simulink model "WaveStar"  (R2018b)
settings: Solver=ode4  StartTime=0  StopTime=141.2  FixedStep=0.001  MaxStep=0.001  RelTol=1e-3  EnableMultiTasking=on
values from neighbouring files (symbols this model uses):
  cc = 10.0    (= 10)    [controller_init.m]
  kc = 0    [controller_init.m]
  L_AB = 0.412    [controller_init.m]
  L_AC = 0.2    [controller_init.m]
  mc = 0    [controller_init.m]
  McSat = inf    [controller_init.m]
  simu = simulationClass()    [wecSimInputFile.m]
  waves = waveClass('irregular')    [wecSimInputFile.m]
  xPcTs = 0.001    [controller_init.m]
undefined symbols (not defined in the file or in its folder): body, constraint, HPfreq, LPfreq, pto, X, Y, Z
libraries: nesl_utility x72, sm_lib x38, WECSim_Lib x7, simulink x2, vrlib x1
(part 3 of 4)

== system WaveStar/Float/Non-Hydro Body/Structure ==
  Total Force : Inport
  Body Properties : sm_lib/Body Elements/Solid  InertiaType=Custom  Mass=body.mass  MassUnits=kg  CenterOfMass=[0 0 0]  CenterOfMassUnits=m  MomentsOfInertia=body.momOfInertia  MomentsOfInertiaUnits=kg*m^2  ProductsOfInertia=[0 0 0]  ProductsOfInertiaUnits=kg*m^2  BasedOnType=Density  Density=1000  DensityUnits=kg/(m^3)  DoExposeReferenceFrame=on  SerializedFrames=<Frames/>  GraphicType=FromGeometry  MarkerShape=Sphere  MarkerSize=10  MarkerSizeUnits=m  GraphicVisPropType=SimpleVisualProperties  GraphicDiffuseColor=body.viz.color  GraphicSpecularColor=[0.5 0.5 0.5 1.0]  GraphicAmbientColor=[0.15 0.15 0.15 1.0]  GraphicEmissiveColor=[0.0 0.0 0.0 1.0]  GraphicShininess=75  GraphicOpacity=body.viz.opacity  GeometryShape=FromFile  RectangleSize=[1 1]  RectangleSizeUnits=m  BrickDimensions=[1 1 1]  BrickDimensionUnits=m  CylinderRadius=1  CylinderRadiusUnits=m  CylinderLength=1  CylinderLengthUnits=m  SphereRadius=1  SphereRadiusUnits=m  EllipsoidRadii=[1 1 1]  EllipsoidRadiiUnits=m  ExtrusionCrossSection=[1 1; -1 1; -1 -1; 1 -1]  ExtrusionCrossSectionUnits=m  ExtrusionLength=1  ExtrusionLengthUnits=m  PolygonNumSides=3  PolygonOuterRadius=1  PolygonOuterRadiusUnits=m  ExtGeomFileType=STL  ExtGeomFileName=geometry/Float.stl  ExtGeomFileUnits=m  RevolutionCrossSection=[1 1; 1 -1; 2 -1; 2 1]  RevolutionCrossSectionUnits=m  RevolutionExtent=Full  RevolutionAngle=180  RevolutionAngleUnits=deg
  External Force and Torque : sm_lib/Forces and Torques/External Force and Torque  ForceResolutionFrame=World  EnableForceX=off  EnableForceY=off  EnableForceZ=off  EnableForce=on  TorqueResolutionFrame=World  EnableTorqueX=off  EnableTorqueY=off  EnableTorqueZ=off  EnableTorque=on
  Motion Sensor : Subsystem
  Rigid Transform (Setup CG) : sm_lib/Frames and Transforms/Rigid Transform  TranslationMethod=Cartesian  TranslationStandardOffset=0  TranslationLengthUnit=m  TranslationStandardAxis=+Z  TranslationCartesianOffset=body.cg  TranslationROffset=0  TranslationROffsetUnits=m  TranslationZOffset=0  TranslationZOffsetUnits=m  TranslationThetaOffset=0  TranslationThetaOffsetUnits=deg  RotationMethod=None  RotationAngleUnits=rad  RotationStandardAxis=+Y  RotationAngle=0.05  RotationArbitraryAxis=[0.57735026918962584 0.57735026918962584 0.57735026918962584]  FollAlignAxisA=+X  BaseAlignAxisA=+Y  FollAlignAxisB=+Y  BaseAlignAxisB=+Z  RotationSequenceAxes=FollowerAxes  RotationSequence=XYX  RotationSequenceAngles=[0 0 0]  RotationSequenceAnglesUnits=deg  RotationMatrix=[1 0 0; 0 1 0; 0 0 1]
  Rigid Transform (Setup Initial Disp) : sm_lib/Frames and Transforms/Rigid Transform  TranslationMethod=Cartesian  TranslationStandardOffset=0  TranslationLengthUnit=m  TranslationStandardAxis=+Z  TranslationCartesianOffset=body.initDisp.initLinDisp  TranslationROffset=0  TranslationROffsetUnits=m  TranslationZOffset=0  TranslationZOffsetUnits=m  TranslationThetaOffset=0  TranslationThetaOffsetUnits=deg  RotationMethod=ArbitraryAxis  RotationAngleUnits=rad  RotationStandardAxis=+Y  RotationAngle=body.initDisp.initAngularDispAngle  RotationArbitraryAxis=body.initDisp.initAngularDispAxis  FollAlignAxisA=+X  BaseAlignAxisA=+Y  FollAlignAxisB=+Y  BaseAlignAxisB=+Z  RotationSequenceAxes=FollowerAxes  RotationSequence=XYX  RotationSequenceAngles=[0 0 0]  RotationSequenceAnglesUnits=deg  RotationMatrix=[1 0 0; 0 1 0; 0 0 1]
  Selector : Selector  InputPortWidth=6  IndexOptions=Index vector (dialog)  Indices=[1:3]  OutputSizes=1
  Selector1 : Selector  InputPortWidth=6  IndexOptions=Index vector (dialog)  Indices=[4:6]  OutputSizes=1
  Simulink-PS Converter1 : nesl_utility/Simulink-PS Converter  PhysicalDomain=network_engine_domain  SubClassName=ps_input  LeftPortType=input  RightPortType=output  PseudoPeriodic=off  Frequencies=[]  NoiseDistribution=none  NoiseParameters=[]  Unit=1  AffineConversion=off  FilteringAndDerivatives=zero  SimscapeFilterOrder=1  InputFilterTimeConstant=0.001  UdotUserProvided=1
  Simulink-PS Converter2 : nesl_utility/Simulink-PS Converter  PhysicalDomain=network_engine_domain  SubClassName=ps_input  LeftPortType=input  RightPortType=output  PseudoPeriodic=off  Frequencies=[]  NoiseDistribution=none  NoiseParameters=[]  Unit=1  AffineConversion=off  FilteringAndDerivatives=zero  SimscapeFilterOrder=1  InputFilterTimeConstant=0.001  UdotUserProvided=1
  World Frame : sm_lib/Frames and Transforms/World Frame
  Conn Free Surface : PMIOPort  Side=Right
  Response : Outport
  wires:
  Total Force/1 -> Selector1/1, Selector/1
  Selector/1 -> Simulink-PS Converter1/1
  Selector1/1 -> Simulink-PS Converter2/1
  Motion Sensor/1(Response) -> Response/1
  connections:
  External Force and Torque/LConn1 -- Simulink-PS Converter1/RConn1
  External Force and Torque/LConn2 -- Simulink-PS Converter2/RConn1
  Rigid Transform (Setup Initial Disp)/RConn1 -- Body Properties/RConn1 -- External Force and Torque/RConn1 -- Motion Sensor/RConn1
  Conn Free Surface/RConn1 -- Rigid Transform (Setup CG)/LConn1
  Rigid Transform (Setup Initial Disp)/LConn1 -- Rigid Transform (Setup CG)/RConn1
  World Frame/RConn1 -- Motion Sensor/LConn1

== system WaveStar/Float/Non-Hydro Body/Weight and Buoyancy ==
  Add1 : Sum  Inputs=+-
  Assignment (Add Net Bouyancy Force to Z-Direction) : Assignment  IndexOptions=Index vector (dialog)  Indices=3  OutputSizes=1
  Body Mass : Constant  Value=body.mass
  Constant1 : Constant  Value=[0 0 0 0 0 0]
  Gravity : Constant  Value=simu.g
  Product : Product
  Product1 : Product  Inputs=3
  Volume : Constant  Value=body.dispVol
  Water Density : Constant  Value=simu.rho
  Out1 : Outport
  wires:
  Add1/1 -> Assignment (Add Net Bouyancy Force to Z-Direction)/2
  Product1/1 -> Add1/2  "F_Buoyancy"
  Product/1 -> Add1/1  "F_Gravity"
  Water Density/1 -> Product1/1  "rho"
  Gravity/1 -> Product/1, Product1/2  "g"
  Volume/1 -> Product1/3  "Vol"
  Assignment (Add Net Bouyancy Force to Z-Direction)/1 -> Out1/1  "F_Restoring"
  Constant1/1 -> Assignment (Add Net Bouyancy Force to Z-Direction)/1
  Body Mass/1 -> Product/2  "m"

== system WaveStar/Controller/Linear/WECCCOMP Controller/lin2rot conversion ==
  float_accel_rot : Inport
  "motor_pos " : Inport  Port=2
  Axial Position : Selector  InputPortWidth=6  IndexOptions=Index vector (dialog)  Indices=[3]  OutputSizes=1
  Constant : Constant  Value=L_AC
  Differentiator with break frequency : DiscreteTransferFcn  Numerator=[1 -1]*2*2*pi*HPfreq.vel  Denominator=[(2+2*pi*HPfreq.vel*xPcTs) (2*pi*HPfreq.vel*xPcTs-2)]
  Divide : Product  Inputs=**
  First order LP filter : DiscreteTransferFcn  Numerator=[1 1]*xPcTs*2*pi*LPfreq.vel  Denominator=[(2+xPcTs*2*pi*LPfreq.vel) (xPcTs*2*pi*LPfreq.vel-2)]
  Linear2Angular Conversion : Subsystem
  Terminator : Terminator
  "float_accel " : Outport
  moment_arm : Outport  Port=2
  motor_vel : Outport  Port=3
  wires:
  "motor_pos "/1 -> Differentiator with break frequency/1, Axial Position/1
  Linear2Angular Conversion/2(moment_arm) -> moment_arm/1
  Axial Position/1 -> Linear2Angular Conversion/1(x_cyl)
  Linear2Angular Conversion/1(Theta) -> Terminator/1
  float_accel_rot/1 -> Divide/1
  Constant/1 -> Divide/2
  Divide/1 -> "float_accel "/1  "Angular Acceleration"
  Differentiator with break frequency/1 -> First order LP filter/1
  First order LP filter/1 -> motor_vel/1

== system WaveStar/Controller/Linear/WECCCOMP Controller/rot2lin conversion ==
  cmd_force_ref : Inport
  moment_arm : Inport  Port=2
  "Divide " : Product  Inputs=*/
  Gain : Gain  Gain=-1
  Multiply : Product  Inputs=**
  Saturation : Saturate  UpperLimit=McSat  LowerLimit=-McSat
  comand torque to measured torque dynamics : DiscreteTransferFcn  Numerator="[ 0.9821   -1.9618    0.9797]"  Denominator="[1.0000   -1.9978    0.9978]"
  cmd_force : Outport
  wires:
  "Divide "/1 -> cmd_force/1
  moment_arm/1 -> Multiply/2, "Divide "/2
  Saturation/1 -> Gain/1  "Mc_sat"
  Gain/1 -> "Divide "/1
  comand torque to measured torque dynamics/1 -> Saturation/1
  cmd_force_ref/1 -> Multiply/1
  Multiply/1 -> comand torque to measured torque dynamics/1

== system WaveStar/Controller/Rotary/lin2rot conversion/Linear2Angular Conversion ==
  x_cyl : Inport
  Divide => K (m) : Product  Inputs=*/
  MATLAB Function1 K [m] : MATLAB Function  TreatAsAtomicUnit=on
  MATLAB Function1 L_BC [m] : MATLAB Function  TreatAsAtomicUnit=on
  MATLAB Function1 Theta [rad] : MATLAB Function  TreatAsAtomicUnit=on
  MATLAB Function1 a_CAB [rad] : MATLAB Function  TreatAsAtomicUnit=on
  Theta : Outport
  moment_arm : Outport  Port=2
  wires:
  MATLAB Function1 L_BC [m]/1(y) -> [L_BC]
  [a_CAB] -> MATLAB Function1 Theta [rad]/1(u)
  MATLAB Function1 K [m]/1(y) -> Divide => K (m)/1
  [L_BC] -> MATLAB Function1 a_CAB [rad]/1(u)
  [L_BC] -> Divide => K (m)/2
  x_cyl/1 -> MATLAB Function1 L_BC [m]/1(u)
  Divide => K (m)/1 -> moment_arm/1
  MATLAB Function1 a_CAB [rad]/1(y) -> [a_CAB]
  [a_CAB] -> MATLAB Function1 K [m]/1(u)
  MATLAB Function1 Theta [rad]/1(y) -> Theta/1

== system WaveStar/Float/Hydrodynamic Body/B2B Subsystem/B2B ==
  CrossCoupling : Subsystem  mask{body=body}
      mask prompts: body "Body Number"
      mask help: This is used to
      mask init:
      | %In the initialization tab we place the code modifying the block
      | 
      | cb = gcb;
      | % position of initial blocks
      | set_param([cb '/vel1'],'Position',[200 1*50 240 (1*50+30)])
      | set_param([cb '/Mux1'], 'Position',[375 40 380 90])
      | set_param([cb '/vel'], 'Position',[410 59 440 71])
      | set_param([cb '/acc1'],'Position',[600 1*50 640 (1*50+30)])
      | set_param([cb '/Mux2'], 'Position',[775 40 780 90])
      | set_param([cb '/acc'], 'Position',[810 59 840 71])
      | 
      | % add/delete lines & blocks
      | newInputs = 0;
      | numbodies = body.bodyTotal;
      | iBod = 2;
      | while iBod < 100
      |     try 
      |         find_system([cb,'/vel',num2str(iBod)],'Type','Block');
      |         if iBod > numbodies
      |             %delete 'From' blocks and lines if bodynumber > total bodies
      |             delete_line(cb,['vel',num2str(iBod),'/1'],['Mux',num2str(1),'/',num2str(iBod)])
      |             delete_line(cb,['acc',num2str(iBod),'/1'],['Mux',num2str(2),'/',num2str(iBod)])
      |             delete_block([cb '/vel',num2str(iBod)])
      |             delete_block([cb '/acc',num2str(iBod)])
      |         end
      |     catch
      |         %set number of outputs for 'Mux Creator' blocks 
      |         if newInputs==0
      |             set_param([cb,'/Mux1'],'Inputs',num2str(numbodies))
      |             set_param([cb,'/Mux2'],'Inputs',num2str(numbodies))
      |         end
      |         if iBod <= numbodies
      |             newInputs = newInputs + 1;
      |             %add velocity 'From' block
      |             add_block('simulink/Signal Routing/From', [cb,'/vel',num2str(iBod)],'MakeNameUnique', 'on',...
      |             'Position',[200 iBod*50 240 (iBod*50+30)], 'BackgroundColor','green')
      |             h=[cb,'/vel',num2str(iBod)];
      |             responseName=['vel' num2str(iBod)];
      |             set_param(h,'GotoTag',responseName);
      |             %add acceleration 'From' block
      |             add_block('simulink/Signal Routing/From', [cb,'/acc',num2str(iBod)],'MakeNameUnique', 'on',...
      |             'Position',[600 iBod*50 640 (iBod*50+30)], 'BackgroundColor','green')
      |             h=[cb,'/acc',num2str(iBod)];
      |             responseName=['acc' num2str(iBod)];
      |             set_param(h,'GotoTag',responseName);
      |             %add lines
      |             add_line(cb,['vel',num2str(iBod),'/1'],['Mux',num2str(1),'/',num2str(iBod)])
      |             add_line(cb,['acc',num2str(iBod),'/1'],['Mux',num2str(2),'/',num2str(iBod)])
      |         else
      |             break
      |         end
      |     end
      |     iBod = iBod + 1;
      | end
      mask Callback body: %customsat_callback('input',gcb)
      mask DialogControl DescGroupVar Prompt: Coupling Block
      mask DialogControl DescTextVar Prompt: This block transfers the velocity and acceleration vectors between bodies allowing for the coupled hydrodynamic forces to be calculated.  This block should not be included if there is only one body or if the hydrodynamic coupling parameter is set to 'No' in the rigid body block.
  vel : Outport
  acc : Outport  Port=2
  wires:
  CrossCoupling/2(acc) -> acc/1
  CrossCoupling/1(vel) -> vel/1

== system WaveStar/Float/Hydrodynamic Body/B2B Subsystem/noB2B ==
  vel_in : Inport
  acc_in : Inport  Port=2
  vel : Outport
  acc : Outport  Port=2
  wires:
  acc_in/1 -> acc/1
  vel_in/1 -> vel/1  "x"

== system WaveStar/Float/Hydrodynamic Body/Hydrostatic Restoring Force Calculation/Linear and Nonlinear Restoring Force Variant Subsystem ==
  note: 1) Add Subsystem or Model blocks as valid variant choices.
      | 2) You cannot connect blocks at this level. At simulation, connectivity is automatically
      | determined, based on the active variant and port name matching.
  In1 : Inport
  In2 : Inport  Port=2
  "Linear Hydrostatic Restoring Force " : Subsystem  VariantControl=sv_linearHydro
  Nonlinear Hydrostatic Restoring Force : Subsystem  VariantControl=sv_nonlinearHydro
  Out1 : Outport

== system WaveStar/Float/Hydrodynamic Body/Morison Element and ViscousDampingForceCalculation/Morison Element Variant Subsystem ==
  note: 1) Add Subsystem or Model blocks as valid variant choices.
      | 2) You cannot connect blocks at this level. At simulation, connectivity is automatically
      | determined, based on the active variant and port name matching.
  displacement : Inport
  velocity : Inport  Port=2
  acceleration : Inport  Port=3
  time : Inport  Port=4
  Morison Element Off : Subsystem  VariantControl=sv_MEOff
  Morison Element On : Subsystem  Variant=on  VariantControl=sv_MEOn
  morison_force : Outport

== system WaveStar/Float/Hydrodynamic Body/Nonlinear Wave Elevation/Linear or Instantaneous Free Surface ==
  note: 1) Add Subsystem or Model blocks as valid variant choices.
      | 2) You cannot connect blocks at this level. At simulation, connectivity is automatically
      | determined, based on the active variant and port name matching.
  In1 : Inport
  In2 : Inport  Port=2
  "Instantaneous Water Free Surface  " : Subsystem  VariantControl=sv_instFS
  "Mean Water Free Surface " : Subsystem  VariantControl=sv_meanFS
  Out1 : Outport

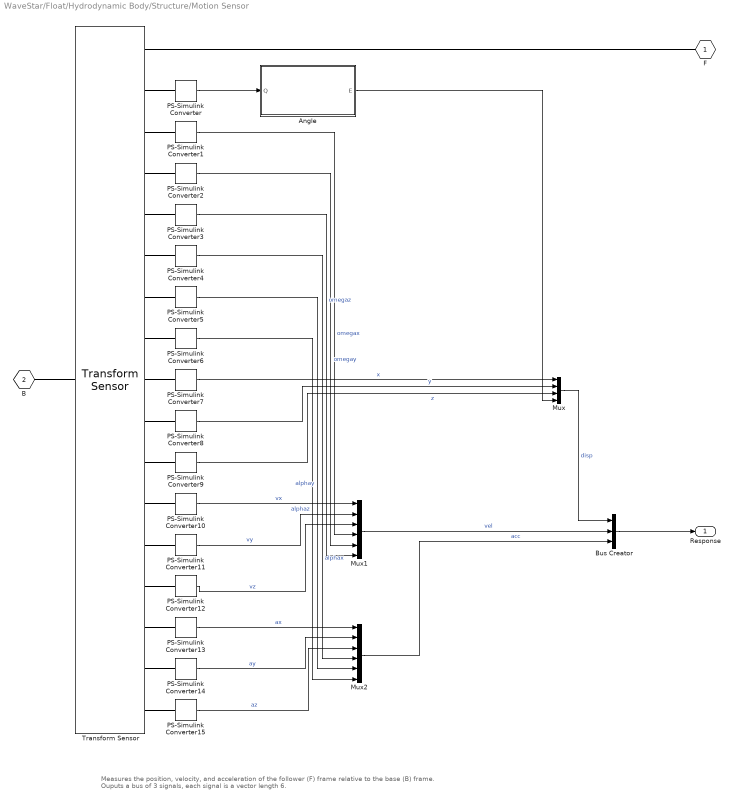
== system WaveStar/Float/Hydrodynamic Body/Structure/Motion Sensor ==
  note: Measures the position, velocity, and acceleration of the follower (F) frame relative to the base (B) frame.
      | Ouputs a bus of 3 signals, each signal is a vector length 6.
  Angle : MATLAB Function  TreatAsAtomicUnit=on
  Bus Creator : BusCreator  Inputs=3
  Mux : Mux
  Mux1 : Mux  Inputs=6
  Mux2 : Mux  Inputs=6
  PS-Simulink Converter{,1..15} (16 alike) : nesl_utility/PS-Simulink Converter  PhysicalDomain=network_engine_domain  SubClassName=ps_output  LeftPortType=input  RightPortType=output  PseudoPeriodic=off  Frequencies=[]  Unit=1  AffineConversion=off
  Transform Sensor : sm_lib/Frames and Transforms/Transform Sensor  MeasurementFrame=World  SenseAngle=off  SenseAxis=off  SenseAngle1=off  SenseAngle2=off  SenseAngle3=off  SenseQ=on  SenseR=off  SenseOmegaX=on  SenseOmegaY=on  SenseOmegaZ=on  SenseOmega1=off  SenseOmega2=off  SenseOmega3=off  SenseQDot=off  SenseRDot=off  SenseAlphaX=on  SenseAlphaY=on  SenseAlphaZ=on  SenseAlpha1=off  SenseAlpha2=off  SenseAlpha3=off  SenseQDDot=off  SenseRDDot=off  SenseX=on  SenseY=on  SenseZ=on  SenseRad=off  SenseAzim=off  SenseDist=off  SenseInc=off  SenseXDot=on  SenseYDot=on  SenseZDot=on  SenseRadDot=off  SenseAzimDot=off  SenseDistDot=off  SenseIncDot=off  SenseXDDot=on  SenseYDDot=on  SenseZDDot=on  SenseRadDDot=off  SenseAzimDDot=off  SenseDistDDot=off  SenseIncDDot=off
  F : PMIOPort  Side=Right
  B : PMIOPort  Port=2  Side=Left
  Response : Outport
  wires:
  PS-Simulink Converter/1 -> Angle/1(Q)
  PS-Simulink Converter4/1 -> Mux2/4  "alphax"
  PS-Simulink Converter10/1 -> Mux1/1  "vx"
  PS-Simulink Converter12/1 -> Mux1/3  "vz"
  PS-Simulink Converter13/1 -> Mux2/1  "ax"
  PS-Simulink Converter14/1 -> Mux2/2  "ay"
  Mux/1 -> Bus Creator/1  "disp"
  Mux1/1 -> Bus Creator/2  "vel"
  Mux2/1 -> Bus Creator/3  "acc"
  Angle/1(E) -> Mux/4
  PS-Simulink Converter7/1 -> Mux/1  "x"
  PS-Simulink Converter8/1 -> Mux/2  "y"
  PS-Simulink Converter9/1 -> Mux/3  "z"
  PS-Simulink Converter5/1 -> Mux2/5  "alphay"
  PS-Simulink Converter6/1 -> Mux2/6  "alphaz"
  PS-Simulink Converter1/1 -> Mux1/4  "omegax"
  PS-Simulink Converter2/1 -> Mux1/5  "omegay"
  PS-Simulink Converter11/1 -> Mux1/2  "vy"
  PS-Simulink Converter3/1 -> Mux1/6  "omegaz"
  PS-Simulink Converter15/1 -> Mux2/3  "az"
  Bus Creator/1 -> Response/1
  connections:
  Transform Sensor/RConn1 -- F/RConn1
  B/RConn1 -- Transform Sensor/LConn1
  Transform Sensor/RConn2 -- PS-Simulink Converter/LConn1
  PS-Simulink Converter15/LConn1 -- Transform Sensor/RConn17
  PS-Simulink Converter14/LConn1 -- Transform Sensor/RConn16
  PS-Simulink Converter13/LConn1 -- Transform Sensor/RConn15
  PS-Simulink Converter12/LConn1 -- Transform Sensor/RConn14
  PS-Simulink Converter11/LConn1 -- Transform Sensor/RConn13
  PS-Simulink Converter10/LConn1 -- Transform Sensor/RConn12
  PS-Simulink Converter9/LConn1 -- Transform Sensor/RConn11
  PS-Simulink Converter8/LConn1 -- Transform Sensor/RConn10
  PS-Simulink Converter7/LConn1 -- Transform Sensor/RConn9
  PS-Simulink Converter4/LConn1 -- Transform Sensor/RConn6
  PS-Simulink Converter5/LConn1 -- Transform Sensor/RConn7
  PS-Simulink Converter6/LConn1 -- Transform Sensor/RConn8
  PS-Simulink Converter1/LConn1 -- Transform Sensor/RConn3
  PS-Simulink Converter2/LConn1 -- Transform Sensor/RConn4
  PS-Simulink Converter3/LConn1 -- Transform Sensor/RConn5

== system WaveStar/Float/Hydrodynamic Body/Wave Diffraction and Excitation Force Calculation/Linear Wave Excitation Force Variant Subsystem ==
  note: 1) Add Subsystem or Model blocks as valid variant choices.
      | 2) You cannot connect blocks at this level. At simulation, connectivity is automatically
      | determined, based on the active variant and port name matching.
  Time : Inport
  Irregular Wave Excitation Force : Subsystem  VariantControl=sv_irregularWaves
  No Wave Excitation Force : Subsystem  VariantControl=sv_noWave
  Regular Wave Excitation Force : Subsystem  VariantControl=sv_regularWaves
  User Defined Wave Excitation Force : Subsystem  VariantControl=sv_udfWaves
  Linear Excitation : Outport

== system WaveStar/Float/Hydrodynamic Body/Wave Diffraction and Excitation Force Calculation/No Ramp Function ==
  Action Port : ActionPort  ActionType=else
  Constant : Constant
  R : Outport  InitialOutput=1
  wires:
  Constant/1 -> R/1

== system WaveStar/Float/Hydrodynamic Body/Wave Diffraction and Excitation Force Calculation/Nonlinear FK Force Variant Subsystem ==
  note: 1) Add Subsystem or Model blocks as valid variant choices.
      | 2) You cannot connect blocks at this level. At simulation, connectivity is automatically
      | determined, based on the active variant and port name matching.
  Time : Inport
  Displacement : Inport  Port=2
  WaveElv : Inport  Port=3
  No Nonlinear FroudeKrylov Force : Subsystem  VariantControl=sv_linearHydro
  With Nonlinear FroudeKrylov Force : Subsystem  TreatAsAtomicUnit=on  SystemSampleTime=simu.dtNL  VariantControl=sv_nonlinearHydro
  Nonlinear Excitation : Outport

== system WaveStar/Float/Hydrodynamic Body/Wave Diffraction and Excitation Force Calculation/Ramp Function ==
  Time : Inport
  Action Port : ActionPort  ActionType=then
  Add : Sum
  Add1 : Sum
  Constant : Constant  Value=1/2
  Constant1 : Constant
  Constant2 : Constant  Value=3*pi/2
  Constant3 : Constant  Value=pi
  Divide : Product  Inputs=*/
  Product : Product
  Product1 : Product
  Ramp Time : Constant  Value=simu.rampTime
  Sine Wave Function : Sin  TimeSource=Use external signal  SampleTime=0
  R : Outport
  wires:
  Divide/1 -> Product1/2  "frequency"
  Constant3/1 -> Divide/1
  Product1/1 -> Add1/1
  Add1/1 -> Sine Wave Function/1
  Constant2/1 -> Add1/2  "phase"
  Ramp Time/1 -> Divide/2  "t_ramp"
  Time/1 -> Product1/1  "t"
  Product/1 -> R/1
  Constant/1 -> Product/2
  Constant1/1 -> Add/1
  Sine Wave Function/1 -> Add/2
  Add/1 -> Product/1

== system WaveStar/Float/Hydrodynamic Body/Wave Radiation Forces Calculation/SS CI and Constant-Damping-CoeVariant Subsystem ==
  note: 1) Add Subsystem or Model blocks as valid variant choices.
      | 2) You cannot connect blocks at this level. At simulation, connectivity is automatically
      | determined, based on the active variant and port name matching.
  In1 : Inport
  In2 : Inport  Port=2
  Constant Coefficients : Subsystem  VariantControl=sv_constantCoeff
  Convolution Integral Calculation : Subsystem  VariantControl=sv_convolution
  "State-Space Calculation " : Subsystem  VariantControl=sv_stateSpace
  Out1 : Outport

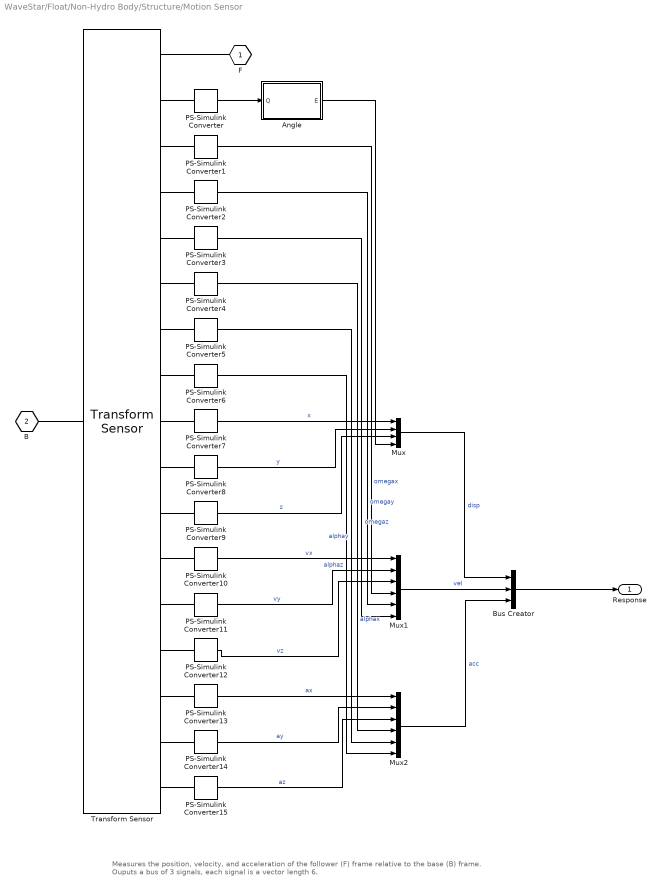
== system WaveStar/Float/Non-Hydro Body/Structure/Motion Sensor ==
  note: Measures the position, velocity, and acceleration of the follower (F) frame relative to the base (B) frame.
      | Ouputs a bus of 3 signals, each signal is a vector length 6.
  Angle : MATLAB Function  TreatAsAtomicUnit=on
  Bus Creator : BusCreator  Inputs=3
  Mux : Mux
  Mux1 : Mux  Inputs=6
  Mux2 : Mux  Inputs=6
  PS-Simulink Converter{,1..15} (16 alike) : nesl_utility/PS-Simulink Converter  PhysicalDomain=network_engine_domain  SubClassName=ps_output  LeftPortType=input  RightPortType=output  PseudoPeriodic=off  Frequencies=[]  Unit=1  AffineConversion=off
  Transform Sensor : sm_lib/Frames and Transforms/Transform Sensor  MeasurementFrame=World  SenseAngle=off  SenseAxis=off  SenseAngle1=off  SenseAngle2=off  SenseAngle3=off  SenseQ=on  SenseR=off  SenseOmegaX=on  SenseOmegaY=on  SenseOmegaZ=on  SenseOmega1=off  SenseOmega2=off  SenseOmega3=off  SenseQDot=off  SenseRDot=off  SenseAlphaX=on  SenseAlphaY=on  SenseAlphaZ=on  SenseAlpha1=off  SenseAlpha2=off  SenseAlpha3=off  SenseQDDot=off  SenseRDDot=off  SenseX=on  SenseY=on  SenseZ=on  SenseRad=off  SenseAzim=off  SenseDist=off  SenseInc=off  SenseXDot=on  SenseYDot=on  SenseZDot=on  SenseRadDot=off  SenseAzimDot=off  SenseDistDot=off  SenseIncDot=off  SenseXDDot=on  SenseYDDot=on  SenseZDDot=on  SenseRadDDot=off  SenseAzimDDot=off  SenseDistDDot=off  SenseIncDDot=off
  F : PMIOPort  Side=Right
  B : PMIOPort  Port=2  Side=Left
  Response : Outport
  wires:
  PS-Simulink Converter/1 -> Angle/1(Q)
  PS-Simulink Converter4/1 -> Mux2/4  "alphax"
  PS-Simulink Converter10/1 -> Mux1/1  "vx"
  PS-Simulink Converter12/1 -> Mux1/3  "vz"
  PS-Simulink Converter13/1 -> Mux2/1  "ax"
  PS-Simulink Converter14/1 -> Mux2/2  "ay"
  Mux/1 -> Bus Creator/1  "disp"
  Mux1/1 -> Bus Creator/2  "vel"
  Mux2/1 -> Bus Creator/3  "acc"
  Angle/1(E) -> Mux/4
  PS-Simulink Converter7/1 -> Mux/1  "x"
  PS-Simulink Converter8/1 -> Mux/2  "y"
  PS-Simulink Converter9/1 -> Mux/3  "z"
  PS-Simulink Converter5/1 -> Mux2/5  "alphay"
  PS-Simulink Converter6/1 -> Mux2/6  "alphaz"
  PS-Simulink Converter1/1 -> Mux1/4  "omegax"
  PS-Simulink Converter2/1 -> Mux1/5  "omegay"
  PS-Simulink Converter11/1 -> Mux1/2  "vy"
  PS-Simulink Converter3/1 -> Mux1/6  "omegaz"
  PS-Simulink Converter15/1 -> Mux2/3  "az"
  Bus Creator/1 -> Response/1
  connections:
  Transform Sensor/RConn1 -- F/RConn1
  B/RConn1 -- Transform Sensor/LConn1
  Transform Sensor/RConn2 -- PS-Simulink Converter/LConn1
  PS-Simulink Converter15/LConn1 -- Transform Sensor/RConn17
  PS-Simulink Converter14/LConn1 -- Transform Sensor/RConn16
  PS-Simulink Converter13/LConn1 -- Transform Sensor/RConn15
  PS-Simulink Converter12/LConn1 -- Transform Sensor/RConn14
  PS-Simulink Converter11/LConn1 -- Transform Sensor/RConn13
  PS-Simulink Converter10/LConn1 -- Transform Sensor/RConn12
  PS-Simulink Converter9/LConn1 -- Transform Sensor/RConn11
  PS-Simulink Converter8/LConn1 -- Transform Sensor/RConn10
  PS-Simulink Converter7/LConn1 -- Transform Sensor/RConn9
  PS-Simulink Converter4/LConn1 -- Transform Sensor/RConn6
  PS-Simulink Converter5/LConn1 -- Transform Sensor/RConn7
  PS-Simulink Converter6/LConn1 -- Transform Sensor/RConn8
  PS-Simulink Converter1/LConn1 -- Transform Sensor/RConn3
  PS-Simulink Converter2/LConn1 -- Transform Sensor/RConn4
  PS-Simulink Converter3/LConn1 -- Transform Sensor/RConn5

== system WaveStar/Controller/Linear/WECCCOMP Controller/lin2rot conversion/Linear2Angular Conversion ==
  x_cyl : Inport
  Divide => K (m) : Product  Inputs=*/
  MATLAB Function1 K [m] : MATLAB Function  TreatAsAtomicUnit=on
  MATLAB Function1 L_BC [m] : MATLAB Function  TreatAsAtomicUnit=on
  MATLAB Function1 Theta [rad] : MATLAB Function  TreatAsAtomicUnit=on
  MATLAB Function1 a_CAB [rad] : MATLAB Function  TreatAsAtomicUnit=on
  Theta : Outport
  moment_arm : Outport  Port=2
  wires:
  MATLAB Function1 L_BC [m]/1(y) -> [L_BC]
  [a_CAB] -> MATLAB Function1 Theta [rad]/1(u)
  MATLAB Function1 K [m]/1(y) -> Divide => K (m)/1
  [L_BC] -> MATLAB Function1 a_CAB [rad]/1(u)
  [L_BC] -> Divide => K (m)/2
  x_cyl/1 -> MATLAB Function1 L_BC [m]/1(u)
  Divide => K (m)/1 -> moment_arm/1
  MATLAB Function1 a_CAB [rad]/1(y) -> [a_CAB]
  [a_CAB] -> MATLAB Function1 K [m]/1(u)
  MATLAB Function1 Theta [rad]/1(y) -> Theta/1

== system WaveStar/Float/Hydrodynamic Body/B2B Subsystem/B2B/CrossCoupling ==
  note: CrossCoupling block is updated by its mask initialization, which is only called on when a simulation is run. 'From' blocks are automatically created and connected based on the number of bodies in the simulation.
  Mux1 : Mux  Inputs=2
  Mux2 : Mux  Inputs=2
  vel : Outport
  acc : Outport  Port=2
  wires:
  [acc2] -> Mux2/2
  Mux2/1 -> acc/1
  [acc1] -> Mux2/1
  [vel2] -> Mux1/2
  Mux1/1 -> vel/1
  [vel1] -> Mux1/1

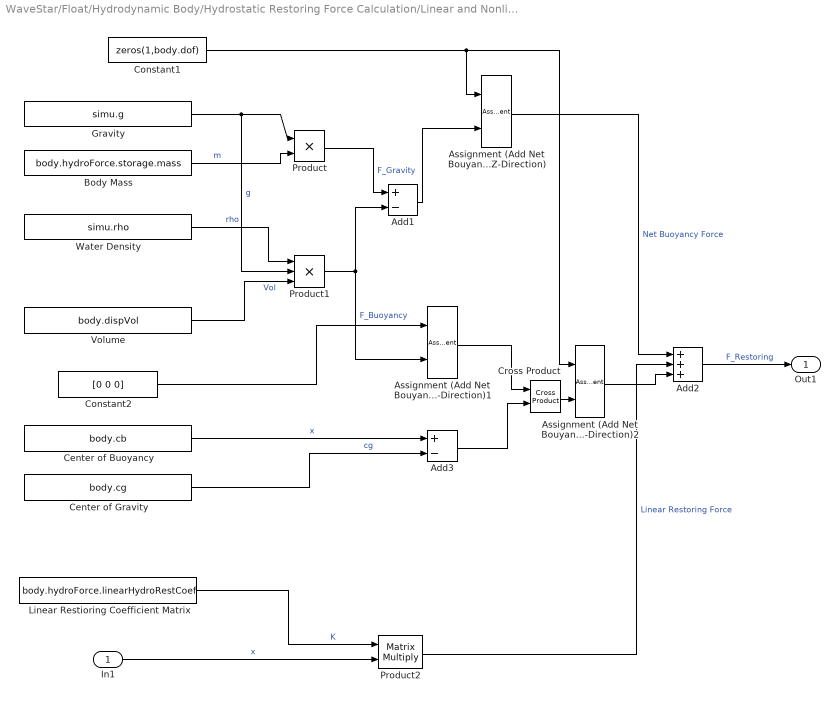
== system WaveStar/Float/Hydrodynamic Body/Hydrostatic Restoring Force Calculation/Linear and Nonlinear Restoring Force Variant Subsystem/Linear Hydrostatic Restoring Force  ==
  In1 : Inport
  Add1 : Sum  Inputs=+-
  Add2 : Sum  Inputs=+++
  Add3 : Sum  Inputs=+-
  Assignment (Add Net Bouyancy Force to Z-Direction) : Assignment  IndexOptions=Index vector (dialog)  Indices=3  OutputSizes=1
  Assignment (Add Net Bouyancy Force to Z-Direction)1 : Assignment  IndexOptions=Index vector (dialog)  Indices=3  OutputSizes=1
  Assignment (Add Net Bouyancy Force to Z-Direction)2 : Assignment  IndexOptions=Index vector (dialog)  Indices=4:6  OutputSizes=1
  Body Mass : Constant  Value=body.hydroForce.storage.mass
  Center of Buoyancy : Constant  Value=body.cb
  Center of Gravity : Constant  Value=body.cg
  Constant1 : Constant  Value=zeros(1,body.dof)
  Constant2 : Constant  Value=[0 0 0]
  Cross Product : vrlib/Utilities/Cross Product
      settings: SourceProductBaseCode=VR
  Gravity : Constant  Value=simu.g
  Linear Restioring Coefficient Matrix : Constant  Value=body.hydroForce.linearHydroRestCoef
  Product : Product
  Product1 : Product  Inputs=3
  Product2 : Product  Multiplication=Matrix(*)
  Volume : Constant  Value=body.dispVol
  Water Density : Constant  Value=simu.rho
  Out1 : Outport
  wires:
  Assignment (Add Net Bouyancy Force to Z-Direction)2/1 -> Add2/3
  Constant1/1 -> Assignment (Add Net Bouyancy Force to Z-Direction)/1, Assignment (Add Net Bouyancy Force to Z-Direction)2/1
  Cross Product/1 -> Assignment (Add Net Bouyancy Force to Z-Direction)2/2
  Assignment (Add Net Bouyancy Force to Z-Direction)1/1 -> Cross Product/1
  Constant2/1 -> Assignment (Add Net Bouyancy Force to Z-Direction)1/1
  Add3/1 -> Cross Product/2
  Center of Gravity/1 -> Add3/2  "cg"
  Center of Buoyancy/1 -> Add3/1  "x"
  Linear Restioring Coefficient Matrix/1 -> Product2/1  "K"
  Product2/1 -> Add2/2  "Linear Restoring Force"
  Add1/1 -> Assignment (Add Net Bouyancy Force to Z-Direction)/2
  Product1/1 -> Assignment (Add Net Bouyancy Force to Z-Direction)1/2, Add1/2  "F_Buoyancy"
  Product/1 -> Add1/1  "F_Gravity"
  Water Density/1 -> Product1/1  "rho"
  Gravity/1 -> Product/1, Product1/2  "g"
  Volume/1 -> Product1/3  "Vol"
  Add2/1 -> Out1/1  "F_Restoring"
  Assignment (Add Net Bouyancy Force to Z-Direction)/1 -> Add2/1  "Net Buoyancy Force"
  Body Mass/1 -> Product/2  "m"
  In1/1 -> Product2/2  "x"

== system WaveStar/Float/Hydrodynamic Body/Hydrostatic Restoring Force Calculation/Linear and Nonlinear Restoring Force Variant Subsystem/Nonlinear Hydrostatic Restoring Force ==
  In1 : Inport
  In2 : Inport  Port=2
  Body Mass2 : Constant  Value=body.hydroForce.storage.mass
  Center of Gravity : Constant  Value=body.cg
  Gravity2 : Constant  Value=simu.g
  Rate Transition : RateTransition
  Rate Transition1 : RateTransition
  Restoring Forces : MATLAB Function  TreatAsAtomicUnit=on  SystemSampleTime=simu.dtNL
  STL areas : Constant  Value=body.bodyGeometry.area
  STL centers : Constant  Value=body.bodyGeometry.center
  STL normal vectors : Constant  Value=body.bodyGeometry.norm
  To Workspace1 : ToWorkspace  VariableName=body1_hspressure_out  SaveFormat=Structure With Time  SampleTime=-1
      settings: Decimation=round(simu.dtOut/simu.dt,0)
  Water Density1 : Constant  Value=simu.rho
  Out1 : Outport
  wires:
  Rate Transition/1 -> Out1/1
  Restoring Forces/1(f) -> Rate Transition/1
  Rate Transition1/1 -> To Workspace1/1
  Restoring Forces/2(p) -> Rate Transition1/1
  Body Mass2/1 -> Restoring Forces/9(mass)
  STL areas/1 -> Restoring Forces/5(area)
  In2/1 -> Restoring Forces/2(elv)
  STL centers/1 -> Restoring Forces/3(center)
  STL normal vectors/1 -> Restoring Forces/4(tnorm)
  Water Density1/1 -> Restoring Forces/6(rho)
  Gravity2/1 -> Restoring Forces/7(g)  "g"
  Center of Gravity/1 -> Restoring Forces/8(cg)
  In1/1 -> Restoring Forces/1(x)

== system WaveStar/Float/Hydrodynamic Body/Morison Element and ViscousDampingForceCalculation/Morison Element Variant Subsystem/Morison Element Off ==
  Constant : Constant  Value=zeros(1,body.dof)
  morison_force : Outport
  wires:
  Constant/1 -> morison_force/1

== system WaveStar/Float/Hydrodynamic Body/Morison Element and ViscousDampingForceCalculation/Morison Element Variant Subsystem/Morison Element On ==
  note: 1) Add Subsystem or Model blocks as valid variant choices.
      | 2) You cannot connect blocks at this level. At simulation, connectivity is automatically
      | determined, based on the active variant and port name matching.
  displacement : Inport
  velocity : Inport  Port=2
  acceleration : Inport  Port=3
  time : Inport  Port=4
  Irregular Wave Morison Force : Subsystem  TreatAsAtomicUnit=on  SystemSampleTime=simu.dtME  VariantControl=sv_irregularWaves
  No Wave Morison Force : Subsystem  VariantControl=sv_noWave
  Regular Wave Morison Force : Subsystem  TreatAsAtomicUnit=on  SystemSampleTime=simu.dtME  VariantControl=sv_regularWaves
  morison_force : Outport

== system WaveStar/Float/Hydrodynamic Body/Nonlinear Wave Elevation/Linear or Instantaneous Free Surface/Instantaneous Water Free Surface   ==
  In1 : Inport
  In2 : Inport  Port=2
  Center of Gravity : Constant  Value=body.cg
  Frequency Spacing : Constant  Value=waves.dw
  Instantaneous FS : MATLAB Function  TreatAsAtomicUnit=on
  Ramp Time : Constant  Value=simu.rampTime
  STL Centers : Constant  Value=body.bodyGeometry.center
  Wave Amplitude : Constant  Value=waves.A
  Wave Direction : Constant  Value=waves.waveDir
  Wave Frequency : Constant  Value=waves.w
  Wave Number : Constant  Value=waves.k
  Wave Random Phase : Constant  Value=waves.phase
  Wave Type Number : Constant  Value=waves.typeNum
  Out1 : Outport
  wires:
  Wave Amplitude/1 -> Instantaneous FS/4(AH)
  Wave Direction/1 -> Instantaneous FS/12(waveDir)
  In1/1 -> Instantaneous FS/1(x)
  In2/1 -> Instantaneous FS/9(t)
  Frequency Spacing/1 -> Instantaneous FS/6(dw)
  Wave Random Phase/1 -> Instantaneous FS/11(phaseRand)
  Ramp Time/1 -> Instantaneous FS/10(rampT)
  Wave Type Number/1 -> Instantaneous FS/8(typeNum)
  Wave Frequency/1 -> Instantaneous FS/5(w)
  Wave Number/1 -> Instantaneous FS/7(k)
  Center of Gravity/1 -> Instantaneous FS/3(cg)
  STL Centers/1 -> Instantaneous FS/2(center)
  Instantaneous FS/1(f) -> Out1/1

== system WaveStar/Float/Hydrodynamic Body/Nonlinear Wave Elevation/Linear or Instantaneous Free Surface/Mean Water Free Surface  ==
  zero : Constant  Value=0
  Out1 : Outport
  wires:
  zero/1 -> Out1/1

== system WaveStar/Float/Hydrodynamic Body/Wave Diffraction and Excitation Force Calculation/Linear Wave Excitation Force Variant Subsystem/Irregular Wave Excitation Force ==
  note: Calculates the wave force, F_wave, for the case of Irregular Waves.
      |
      | F_wave = sum( F_wave(i))
      |
      | where i = each frequency bin.
  Time : Inport
  Frequency Spacing Delta Omega : Constant  Value=waves.dw  VectorParams1D=off
  Imaginary Part of Wave Excitation : Constant  Value=body.hydroForce.fExt.im  VectorParams1D=off
  MATLAB Function : MATLAB Function  TreatAsAtomicUnit=on
  Random Phase : Constant  Value=waves.phase  VectorParams1D=off
  Real Part of Wave Excitation : Constant  Value=body.hydroForce.fExt.re  VectorParams1D=off
  Real Part of Wave Excitation1 : Constant  Value=body.hydroForce.fExt.md  VectorParams1D=off
  Wave Frequency : Constant  Value=waves.w  VectorParams1D=off
  Wave Spectrum : Constant  Value=waves.A  VectorParams1D=off
  Wave direction : Constant  Value=waves.waveDir  VectorParams1D=off
  Wave direction spread : Constant  Value=waves.waveSpread  VectorParams1D=off
  Linear Excitation : Outport
  wires:
  Real Part of Wave Excitation1/1 -> MATLAB Function/10(fExtMD)
  Wave direction/1 -> MATLAB Function/8(WaveDir)
  Wave direction spread/1 -> MATLAB Function/9(WaveSpread)
  Frequency Spacing Delta Omega/1 -> MATLAB Function/6(dw)
  Time/1 -> MATLAB Function/7(time)
  Wave Spectrum/1 -> MATLAB Function/1(A)
  Real Part of Wave Excitation/1 -> MATLAB Function/3(fExtRE)
  Imaginary Part of Wave Excitation/1 -> MATLAB Function/4(fExtIM)
  Wave Frequency/1 -> MATLAB Function/2(w)
  MATLAB Function/1(Fext) -> Linear Excitation/1
  Random Phase/1 -> MATLAB Function/5(phaseRand)

== system WaveStar/Float/Hydrodynamic Body/Wave Diffraction and Excitation Force Calculation/Linear Wave Excitation Force Variant Subsystem/No Wave Excitation Force ==
  Constant : Constant  Value=zeros(1,body.dof)
  Linear Excitation : Outport
  wires:
  Constant/1 -> Linear Excitation/1

== system WaveStar/Float/Hydrodynamic Body/Wave Diffraction and Excitation Force Calculation/Linear Wave Excitation Force Variant Subsystem/Regular Wave Excitation Force ==
  note: Calculates the wave force, F_wave, for the case of Regular Waves.
      |
      | F_wave =   A * cos(w * t) * Re{Fext}
      |                -  A * sin(w * t) * Im{Fext}
  Time : Inport
  Add : Sum
  Add1 : Sum  Inputs=++-
  Constant : Constant  Value=pi/2
  Excitation Imaginary Part : Constant  Value=body.hydroForce.fExt.im(1,:)  VectorParams1D=off
  Excitation Real Part : Constant  Value=body.hydroForce.fExt.re(1,:)  VectorParams1D=off
  Excitation Real Part1 : Constant  Value=body.hydroForce.fExt.md(1,:)  VectorParams1D=off
  Product : Product
  Product1 : Product  Inputs=3
  Product2 : Product  Inputs=3
  Product3 : Product
  Sine Wave Function : Sin  TimeSource=Use external signal  SampleTime=0
  Sine Wave Function1 : Sin  TimeSource=Use external signal  SampleTime=0
  Wave Amplitude : Constant  Value=waves.A(1,:)
  Wave Amplitude1 : Constant  Value=waves.A(1,:).*waves.A(1,:)
  Wave Frequency : Constant  Value=waves.w(1,:)
  Linear Excitation : Outport
  wires:
  Product3/1 -> Add1/1
  Excitation Real Part1/1 -> Product3/2  "Re{Fext}"
  Wave Amplitude1/1 -> Product3/1  "A"
  Constant/1 -> Add/2
  Add/1 -> Sine Wave Function1/1
  Wave Amplitude/1 -> Product1/1, Product2/1  "A"
  Add1/1 -> Linear Excitation/1
  Product2/1 -> Add1/3
  Product1/1 -> Add1/2
  Excitation Real Part/1 -> Product1/2  "Re{Fext}"
  Excitation Imaginary Part/1 -> Product2/3  "Im{Fext}"
  Sine Wave Function/1 -> Product2/2  "sin(wt)"
  Sine Wave Function1/1 -> Product1/3  "cos(w*t)"
  Product/1 -> Add/1, Sine Wave Function/1
  Wave Frequency/1 -> Product/2  "w"
  Time/1 -> Product/1  "t"

== system WaveStar/Float/Hydrodynamic Body/Wave Diffraction and Excitation Force Calculation/Linear Wave Excitation Force Variant Subsystem/User Defined Wave Excitation Force ==
  note: Calculates the wave force, F_wave, for the case of User Defined Waves.
      |
      | F_wave = convolution calculation [1x6]
  InputWaveForceTimeHistory : FromWorkspace  VariableName=[waves.waveAmpTime(:,1),body.hydroForce.userDefinedFe]  SampleTime=0
  Linear Excitation : Outport
  wires:
  InputWaveForceTimeHistory/1 -> Linear Excitation/1

== system WaveStar/Float/Hydrodynamic Body/Wave Diffraction and Excitation Force Calculation/Nonlinear FK Force Variant Subsystem/No Nonlinear FroudeKrylov Force ==
  Constant : Constant  Value=zeros(1,body.dof)
  Nonlinear Excitation : Outport
  wires:
  Constant/1 -> Nonlinear Excitation/1

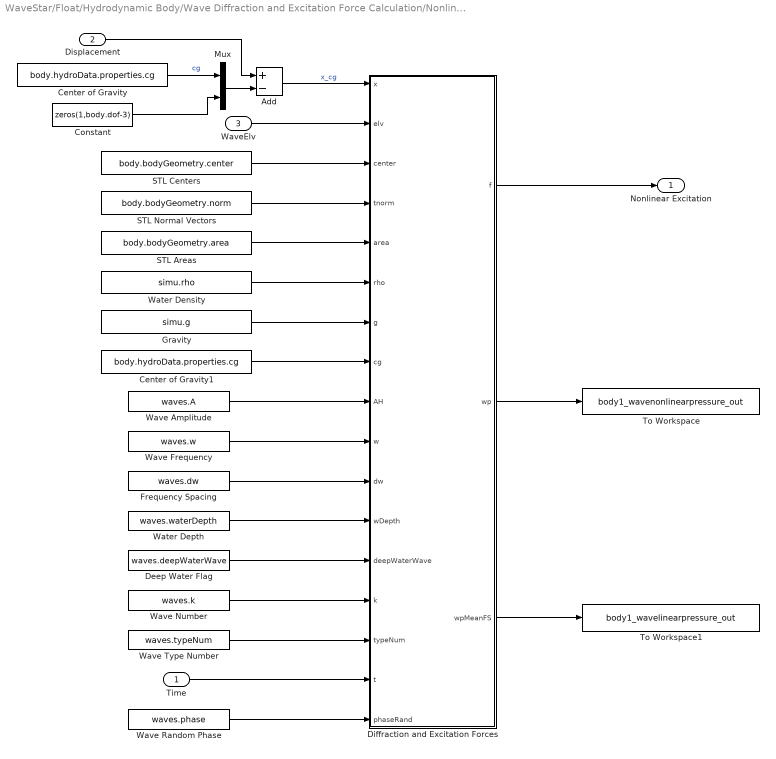
== system WaveStar/Float/Hydrodynamic Body/Wave Diffraction and Excitation Force Calculation/Nonlinear FK Force Variant Subsystem/With Nonlinear FroudeKrylov Force ==
  Time : Inport
  Displacement : Inport  Port=2
  WaveElv : Inport  Port=3
  Add : Sum  Inputs=+-
  Center of Gravity : Constant  Value=body.hydroData.properties.cg
  Center of Gravity1 : Constant  Value=body.hydroData.properties.cg
  Constant : Constant  Value=zeros(1,body.dof-3)
  Deep Water Flag : Constant  Value=waves.deepWaterWave
  Diffraction and Excitation Forces : MATLAB Function  TreatAsAtomicUnit=on
  Frequency Spacing : Constant  Value=waves.dw
  Gravity : Constant  Value=simu.g
  Mux : Mux  Inputs=2
  STL Areas : Constant  Value=body.bodyGeometry.area
  STL Centers : Constant  Value=body.bodyGeometry.center
  STL Normal Vectors : Constant  Value=body.bodyGeometry.norm
  To Workspace : ToWorkspace  VariableName=body1_wavenonlinearpressure_out  SaveFormat=Structure With Time  SampleTime=-1
      settings: Decimation=round(simu.dtOut/simu.dt,0)
  To Workspace1 : ToWorkspace  VariableName=body1_wavelinearpressure_out  SaveFormat=Structure With Time  SampleTime=-1
      settings: Decimation=round(simu.dtOut/simu.dt,0)
  Water Density : Constant  Value=simu.rho
  Water Depth : Constant  Value=waves.waterDepth
  Wave Amplitude : Constant  Value=waves.A
  Wave Frequency : Constant  Value=waves.w
  Wave Number : Constant  Value=waves.k
  Wave Random Phase : Constant  Value=waves.phase
  Wave Type Number : Constant  Value=waves.typeNum
  Nonlinear Excitation : Outport
  wires:
  STL Areas/1 -> Diffraction and Excitation Forces/5(area)
  Diffraction and Excitation Forces/2(wp) -> To Workspace/1
  Diffraction and Excitation Forces/3(wpMeanFS) -> To Workspace1/1
  Displacement/1 -> Add/1
  Constant/1 -> Mux/2
  Center of Gravity/1 -> Mux/1  "cg"
  Mux/1 -> Add/2
  Add/1 -> Diffraction and Excitation Forces/1(x)  "x_cg"
  Deep Water Flag/1 -> Diffraction and Excitation Forces/13(deepWaterWave)
  Wave Random Phase/1 -> Diffraction and Excitation Forces/17(phaseRand)
  Water Depth/1 -> Diffraction and Excitation Forces/12(wDepth)
  Wave Number/1 -> Diffraction and Excitation Forces/14(k)
  Wave Type Number/1 -> Diffraction and Excitation Forces/15(typeNum)
  Frequency Spacing/1 -> Diffraction and Excitation Forces/11(dw)
  Wave Frequency/1 -> Diffraction and Excitation Forces/10(w)
  Wave Amplitude/1 -> Diffraction and Excitation Forces/9(AH)
  Time/1 -> Diffraction and Excitation Forces/16(t)
  WaveElv/1 -> Diffraction and Excitation Forces/2(elv)
  STL Centers/1 -> Diffraction and Excitation Forces/3(center)
  STL Normal Vectors/1 -> Diffraction and Excitation Forces/4(tnorm)
  Water Density/1 -> Diffraction and Excitation Forces/6(rho)
  Gravity/1 -> Diffraction and Excitation Forces/7(g)
  Diffraction and Excitation Forces/1(f) -> Nonlinear Excitation/1
  Center of Gravity1/1 -> Diffraction and Excitation Forces/8(cg)

== system WaveStar/Float/Hydrodynamic Body/Wave Radiation Forces Calculation/SS CI and Constant-Damping-CoeVariant Subsystem/Constant Coefficients ==
  In1 : Inport
  Product : Product  Multiplication=Matrix(*)
  Radiation Damping Matrix : Constant  Value=body.hydroForce.fDamping
  Out1 : Outport
  wires:
  In1/1 -> Product/2
  Product/1 -> Out1/1  "F_Single Frequency"
  Radiation Damping Matrix/1 -> Product/1

== system WaveStar/Float/Hydrodynamic Body/Wave Radiation Forces Calculation/SS CI and Constant-Damping-CoeVariant Subsystem/Convolution Integral Calculation ==
  In1 : Inport
  CTTime : Constant  Value=simu.CTTime
  DOF : Constant  Value=body.dof
  IRBK : Constant  Value=body.hydroForce.irkb
  MATLAB Function1 : MATLAB Function  TreatAsAtomicUnit=on  SystemSampleTime=simu.CTTime(2)-simu.CTTime(1)
  Rate Transition : RateTransition
  Reshape : Reshape
  Out1 : Outport
  wires:
  CTTime/1 -> MATLAB Function1/4(CTTime)
  DOF/1 -> MATLAB Function1/3(lenJ)
  IRBK/1 -> MATLAB Function1/2(IRKB)
  In1/1 -> MATLAB Function1/1(v)
  MATLAB Function1/1(F_FM) -> Rate Transition/1
  Rate Transition/1 -> Reshape/1
  Reshape/1 -> Out1/1

== system WaveStar/Float/Hydrodynamic Body/Wave Radiation Forces Calculation/SS CI and Constant-Damping-CoeVariant Subsystem/State-Space Calculation  ==
  In1 : Inport
  State-Space : StateSpace  A=body.hydroForce.ssRadf.A  B=body.hydroForce.ssRadf.B  C=body.hydroForce.ssRadf.C  D=body.hydroForce.ssRadf.D  InitialCondition=0
  Out1 : Outport
  wires:
  State-Space/1 -> Out1/1
  In1/1 -> State-Space/1  "x"

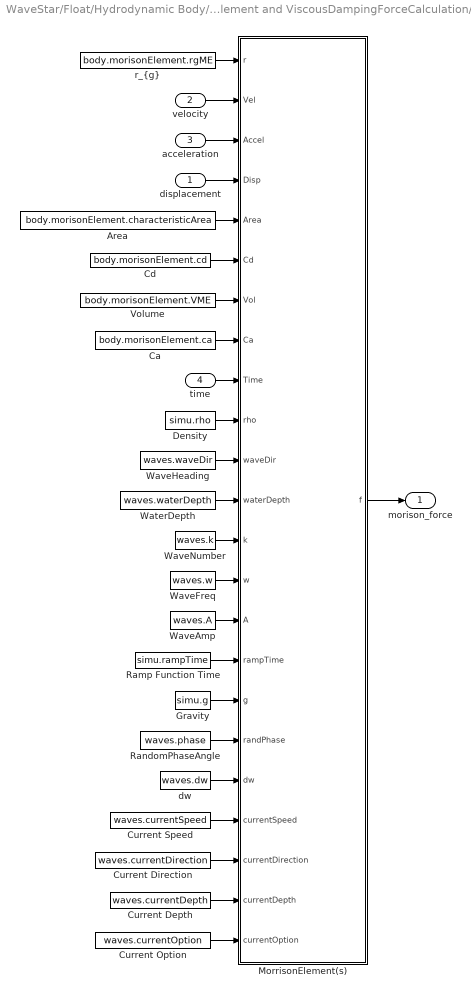
== system WaveStar/Float/Hydrodynamic Body/Morison Element and ViscousDampingForceCalculation/Morison Element Variant Subsystem/Morison Element On/Irregular Wave Morison Force ==
  displacement : Inport
  velocity : Inport  Port=2
  acceleration : Inport  Port=3
  time : Inport  Port=4
  Area : Constant  Value=body.morisonElement.characteristicArea  VectorParams1D=off
  Ca : Constant  Value=body.morisonElement.ca  VectorParams1D=off
  Cd : Constant  Value=body.morisonElement.cd  VectorParams1D=off
  Current Depth : Constant  Value=waves.currentDepth
  Current Direction : Constant  Value=waves.currentDirection
  Current Option : Constant  Value=waves.currentOption
  Current Speed : Constant  Value=waves.currentSpeed
  Density : Constant  Value=simu.rho
  Gravity : Constant  Value=simu.g
  "MorrisonElement(s) " : MATLAB Function  TreatAsAtomicUnit=on
  Ramp Function Time : Constant  Value=simu.rampTime
  RandomPhaseAngle : Constant  Value=waves.phase  VectorParams1D=off
  Volume : Constant  Value=body.morisonElement.VME  VectorParams1D=off
  WaterDepth : Constant  Value=waves.waterDepth
  WaveAmp : Constant  Value=waves.A
  WaveFreq : Constant  Value=waves.w
  WaveHeading : Constant  Value=waves.waveDir
  WaveNumber : Constant  Value=waves.k
  dw : Constant  Value=waves.dw  VectorParams1D=off
  "r_{g}" : Constant  Value=body.morisonElement.rgME  VectorParams1D=off
  morison_force : Outport
  wires:
  "MorrisonElement(s) "/1(f) -> morison_force/1
  Current Option/1 -> "MorrisonElement(s) "/23(currentOption)
  Current Depth/1 -> "MorrisonElement(s) "/22(currentDepth)
  Current Speed/1 -> "MorrisonElement(s) "/20(currentSpeed)
  Current Direction/1 -> "MorrisonElement(s) "/21(currentDirection)
  time/1 -> "MorrisonElement(s) "/9(Time)
  Volume/1 -> "MorrisonElement(s) "/7(Vol)
  acceleration/1 -> "MorrisonElement(s) "/3(Accel)
  displacement/1 -> "MorrisonElement(s) "/4(Disp)
  Area/1 -> "MorrisonElement(s) "/5(Area)
  "r_{g}"/1 -> "MorrisonElement(s) "/1(r)
  velocity/1 -> "MorrisonElement(s) "/2(Vel)
  WaterDepth/1 -> "MorrisonElement(s) "/12(waterDepth)
  Gravity/1 -> "MorrisonElement(s) "/17(g)
  WaveNumber/1 -> "MorrisonElement(s) "/13(k)
  WaveHeading/1 -> "MorrisonElement(s) "/11(waveDir)
  Density/1 -> "MorrisonElement(s) "/10(rho)
  RandomPhaseAngle/1 -> "MorrisonElement(s) "/18(randPhase)
  WaveFreq/1 -> "MorrisonElement(s) "/14(w)
  Ca/1 -> "MorrisonElement(s) "/8(Ca)
  dw/1 -> "MorrisonElement(s) "/19(dw)
  WaveAmp/1 -> "MorrisonElement(s) "/15(A)
  Cd/1 -> "MorrisonElement(s) "/6(Cd)
  Ramp Function Time/1 -> "MorrisonElement(s) "/16(rampTime)

== system WaveStar/Float/Hydrodynamic Body/Morison Element and ViscousDampingForceCalculation/Morison Element Variant Subsystem/Morison Element On/No Wave Morison Force ==
  displacement : Inport
  velocity : Inport  Port=2
  acceleration : Inport  Port=3
  time : Inport  Port=4
  Area : Constant  Value=body.morisonElement.characteristicArea  VectorParams1D=off
  Ca : Constant  Value=body.morisonElement.ca  VectorParams1D=off
  Cd : Constant  Value=body.morisonElement.cd  VectorParams1D=off
  Current Depth : Constant  Value=waves.currentDepth
  Current Direction : Constant  Value=waves.currentDirection
  Current Option : Constant  Value=waves.currentOption
  Current Speed : Constant  Value=waves.currentSpeed
  Density : Constant  Value=simu.rho
  "MorrisonElement(s) " : MATLAB Function  TreatAsAtomicUnit=on
  Ramp Function Time : Constant  Value=simu.rampTime
  Volume : Constant  Value=body.morisonElement.VME  VectorParams1D=off
  "r_{g}" : Constant  Value=body.morisonElement.rgME  VectorParams1D=off
  morison_force : Outport
  wires:
  Current Depth/1 -> "MorrisonElement(s) "/14(currentDepth)
  Current Option/1 -> "MorrisonElement(s) "/15(currentOption)
  Current Speed/1 -> "MorrisonElement(s) "/10(currentSpeed)
  time/1 -> "MorrisonElement(s) "/12(Time)
  Ramp Function Time/1 -> "MorrisonElement(s) "/13(rampTime)
  Current Direction/1 -> "MorrisonElement(s) "/11(currentDirection)
  "MorrisonElement(s) "/1(f) -> morison_force/1
  acceleration/1 -> "MorrisonElement(s) "/3(Accel)
  Density/1 -> "MorrisonElement(s) "/9(rho)
  Volume/1 -> "MorrisonElement(s) "/7(Vol)
  "r_{g}"/1 -> "MorrisonElement(s) "/1(r)
  Ca/1 -> "MorrisonElement(s) "/8(Ca)
  Area/1 -> "MorrisonElement(s) "/5(Area)
  displacement/1 -> "MorrisonElement(s) "/4(Disp)
  Cd/1 -> "MorrisonElement(s) "/6(Cd)
  velocity/1 -> "MorrisonElement(s) "/2(Vel)

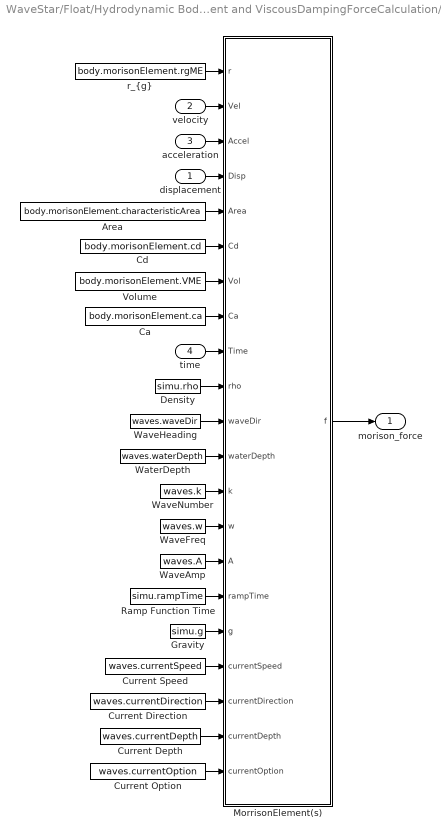
== system WaveStar/Float/Hydrodynamic Body/Morison Element and ViscousDampingForceCalculation/Morison Element Variant Subsystem/Morison Element On/Regular Wave Morison Force ==
  displacement : Inport
  velocity : Inport  Port=2
  acceleration : Inport  Port=3
  time : Inport  Port=4
  Area : Constant  Value=body.morisonElement.characteristicArea  VectorParams1D=off
  Ca : Constant  Value=body.morisonElement.ca  VectorParams1D=off
  Cd : Constant  Value=body.morisonElement.cd  VectorParams1D=off
  Current Depth : Constant  Value=waves.currentDepth
  Current Direction : Constant  Value=waves.currentDirection
  Current Option : Constant  Value=waves.currentOption
  Current Speed : Constant  Value=waves.currentSpeed
  Density : Constant  Value=simu.rho
  Gravity : Constant  Value=simu.g
  "MorrisonElement(s) " : MATLAB Function  TreatAsAtomicUnit=on
  Ramp Function Time : Constant  Value=simu.rampTime
  Volume : Constant  Value=body.morisonElement.VME  VectorParams1D=off
  WaterDepth : Constant  Value=waves.waterDepth
  WaveAmp : Constant  Value=waves.A
  WaveFreq : Constant  Value=waves.w
  WaveHeading : Constant  Value=waves.waveDir
  WaveNumber : Constant  Value=waves.k
  "r_{g}" : Constant  Value=body.morisonElement.rgME  VectorParams1D=off
  morison_force : Outport
  wires:
  Current Depth/1 -> "MorrisonElement(s) "/20(currentDepth)
  Current Option/1 -> "MorrisonElement(s) "/21(currentOption)
  Current Direction/1 -> "MorrisonElement(s) "/19(currentDirection)
  Current Speed/1 -> "MorrisonElement(s) "/18(currentSpeed)
  Ramp Function Time/1 -> "MorrisonElement(s) "/16(rampTime)
  time/1 -> "MorrisonElement(s) "/9(Time)
  "MorrisonElement(s) "/1(f) -> morison_force/1
  Volume/1 -> "MorrisonElement(s) "/7(Vol)
  Ca/1 -> "MorrisonElement(s) "/8(Ca)
  Gravity/1 -> "MorrisonElement(s) "/17(g)
  Cd/1 -> "MorrisonElement(s) "/6(Cd)
  displacement/1 -> "MorrisonElement(s) "/4(Disp)
  WaveAmp/1 -> "MorrisonElement(s) "/15(A)
  WaveFreq/1 -> "MorrisonElement(s) "/14(w)
  Density/1 -> "MorrisonElement(s) "/10(rho)
  acceleration/1 -> "MorrisonElement(s) "/3(Accel)
  velocity/1 -> "MorrisonElement(s) "/2(Vel)
  WaveHeading/1 -> "MorrisonElement(s) "/11(waveDir)
  WaveNumber/1 -> "MorrisonElement(s) "/13(k)
  WaterDepth/1 -> "MorrisonElement(s) "/12(waterDepth)
  "r_{g}"/1 -> "MorrisonElement(s) "/1(r)
  Area/1 -> "MorrisonElement(s) "/5(Area)

== matlab function WaveStar/Controller/Linear/WECCCOMP Controller/lin2rot conversion/Linear2Angular Conversion/MATLAB Function1 K [m] ==
  data: u input; y output; L_AB parameter; L_AC parameter
function y = fcn(u,L_AB,L_AC)
%#codegen
y = L_AB'*L_AC'*sin(u);

== matlab function WaveStar/Controller/Linear/WECCCOMP Controller/lin2rot conversion/Linear2Angular Conversion/MATLAB Function1 L_BC [m] ==
  data: u input; y output; L_BC_neutral parameter
 function y = fcn(u,L_BC_neutral)
%#codegen
%
y = u+L_BC_neutral';

== matlab function WaveStar/Controller/Linear/WECCCOMP Controller/lin2rot conversion/Linear2Angular Conversion/MATLAB Function1 Theta [rad] ==
  data: u input; y output; a_CAB_neutral parameter
function y = fcn(u,a_CAB_neutral)
%#codegen
y = u-a_CAB_neutral';
